simulink model "Bossi_Emanuele_EE460S3D_R99"  (R2025a)
settings: Solver=FixedStepDiscrete  StartTime=0.0  StopTime=120  FixedStep=dt0  RelTol=1e-3  EnableMultiTasking=on
PostLoadFcn:
  | %Set the size for the model
  | set_param(gcs,'Location',[10 10 1270 970])
  | %Set the zoom factor for the model
  | set_param(gcs,'ZoomFactor','100')
InitFcn:
  | tic
  | Bossi_Emanuele_EE460_Final
  | INIT_S3D_01
StartFcn:
  | tend0=toc;
  | tic;
StopFcn:
  | tend=toc;
  | disp(['Simulation time = ' num2str(tout(end)) ' sec'])
  | disp(['Real time = ' num2str(tend) ' sec'])
  | title('DONE')
  | SCORE=round((max(0,120-tout(end)-tend0))*4+10*(40-FuelBurned)+sum(100*double(PDONE)-100*double(PDONE<.5)));
  | PlotS3D(PlotInput);
  | text(15,22,['S: ' num2str(SCORE)]);
  | % Reset color scheme back to normal defaults
  | figure()
  | blkwhitebg('w');
  | close
values from neighbouring files (symbols this model uses):
  A_obs = [ 0  1  0  0  0  0 ... (first row only)    [Bossi_Emanuele_EE460_Final.m]
  B_obs = [ 0     0     0 ... (first row only)    [Bossi_Emanuele_EE460_Final.m]
  C_obs = [ 1 0 0 0 0 0 ... (first row only)    [Bossi_Emanuele_EE460_Final.m]
  d2r = pi/180    (= 0.0174532925199)    [INIT_S3D_01.m]
  D_obs = [ 0     0     0 ... (first row only)    [Bossi_Emanuele_EE460_Final.m]
  dt = 0.01    [INIT_S3D_01.m]
  dt0 = 0.001    [INIT_S3D_01.m]
  fr = 100    [INIT_S3D_01.m]
  G = [1,  1, -1, -1,  0,  0,  0,  0 ... (first row only)    [Bossi_Emanuele_EE460_Final.m]
  G_obs = eye(6)    [Bossi_Emanuele_EE460_Final.m]
  HM_S = 250    [INIT_S3D_01.m]
  HM_U = 500    [INIT_S3D_01.m]
  J = Jbase+JC0+JF+M*(Xcg^2+Ycg^2)    [INIT_S3D_01.m]
  Jbase = JC1+4*Ja+2*Ma*da^2+2*Ma*db^2    [INIT_S3D_01.m]
  JC0 = MC0/2    (= 10.2101761242)    [INIT_S3D_01.m]
  Kdtheta = 2 * zeta_th * wn_th * J_eff    [Bossi_Emanuele_EE460_Final.m]
  Kdtheta_fail = 2 * zeta_th_fail * wn_th_fail * J_eff    [Bossi_Emanuele_EE460_Final.m]
  Kdx = 2 * zeta_xy * wn_xy * M_eff    [Bossi_Emanuele_EE460_Final.m]
  Kdx_fail = 2 * zeta_xy_fail * wn_xy_fail * M_eff    [Bossi_Emanuele_EE460_Final.m]
  Kdy = 2 * zeta_xy * wn_xy * M_eff    [Bossi_Emanuele_EE460_Final.m]
  Kdy_fail = 2 * zeta_xy_fail * wn_xy_fail * M_eff    [Bossi_Emanuele_EE460_Final.m]
  Kptheta = J_eff * wn_th^2    [Bossi_Emanuele_EE460_Final.m]
  Kptheta_fail = J_eff * wn_th_fail^2    [Bossi_Emanuele_EE460_Final.m]
  Kpx = M_eff * wn_xy^2    [Bossi_Emanuele_EE460_Final.m]
  Kpx_fail = M_eff * wn_xy_fail^2    [Bossi_Emanuele_EE460_Final.m]
  Kpy = M_eff * wn_xy^2    [Bossi_Emanuele_EE460_Final.m]
  Kpy_fail = M_eff * wn_xy_fail^2    [Bossi_Emanuele_EE460_Final.m]
  L13 = sqrt(10)    [INIT_S3D_01.m]
  L24 = sqrt(6.25)    [INIT_S3D_01.m]
  LVL = LVL12    [INIT_S3D_01.m]
  M = MC+M1+M2+M3+M4+4*Ma    [INIT_S3D_01.m]
  M1 = LVL.M1    [INIT_S3D_01.m]
  M2 = LVL.M2    [INIT_S3D_01.m]
  M3 = LVL.M3    [INIT_S3D_01.m]
  M4 = LVL.M4    [INIT_S3D_01.m]
  max_qddot = [max_qddot_x; max_qddot_y; max_qddot_theta]    [Bossi_Emanuele_EE460_Final.m]
  mdti = (1/300)    (= 0.00333333333333)    [INIT_S3D_01.m]
  P = [1  1 -1 -1  0  0  0  0 ... (first row only)    [Bossi_Emanuele_EE460_Final.m]
  Pdata = [LVL.P1 LVL.P2 LVL.P3 LVL.P4]    [INIT_S3D_01.m]    (also in PlotS3D.m = R*[xt1;yt1+[0 3*tt*TV(idx-13)*TSIG(idx-13) 0]])
  PTvec = [Pdata(:,1);Pdata(:,2);Pdata(:,3);Pdata(:,4) ... (first row only)    [INIT_S3D_01.m]
  Q_obs = eye(6)    [Bossi_Emanuele_EE460_Final.m]
  r2d = 180/pi    (= 57.2957795131)    [INIT_S3D_01.m]
  r_bang = 0.5    [Bossi_Emanuele_EE460_Final.m]
  Sconfig = 1    [Bossi_Emanuele_EE460_Final.m]
  SLIM = [-100 100 ... (first row only)    [INIT_S3D_01.m]
  SQ = [.005 .01 .004 .005 .01 .004 .02 .01 .4]'    [INIT_S3D_01.m]
  SSF = 1./SQ    [INIT_S3D_01.m]
  tau = 0.5    [Bossi_Emanuele_EE460_Final.m]
  TOLdata = [LVL.P1tol LVL.P2tol LVL.P3tol LVL.P4tol]    [INIT_S3D_01.m]
  ULIM = [[Umin Umax];0 0;0 0]    [INIT_S3D_01.m]
undefined symbols (not defined in the file or in its folder): den_lp, den_lp2, DiscIntNeverNeededParam, dt1_bang_3, dt2_bang_3, dtc_bang_3, num_lp, num_lp2, q0_1
libraries: simulink x87, matrix_library x4, sl3dlib x1, aerolibutil x1, aerolibanimutils x1
(part 7 of 8)

== system Bossi_Emanuele_EE460S3D_R99/S3D_Plant/Sensors/CASE1/THTaccel/CURRENT ==
  In1 : Inport
  Action Port : ActionPort  ActionPortLabel=else
  Out1 : Outport
  wires:
  In1/1 -> Out1/1

== system Bossi_Emanuele_EE460S3D_R99/S3D_Plant/Sensors/CASE1/THTaccel/MAX ==
  Action Port : ActionPort  ActionPortLabel=elseif(u1 > 0.5 & u1 < 1.5)
  Constant : Constant  Value=SLIM(9,2)  SampleTime=dt0
  Out1 : Outport
  wires:
  Constant/1 -> Out1/1

== system Bossi_Emanuele_EE460S3D_R99/S3D_Plant/Sensors/CASE1/THTaccel/MIN ==
  Action Port : ActionPort  ActionPortLabel=if(u1 < -0.5)
  Constant : Constant  Value=SLIM(9,1)  SampleTime=dt0
  Out1 : Outport
  wires:
  Constant/1 -> Out1/1

== system Bossi_Emanuele_EE460S3D_R99/S3D_Plant/Sensors/CASE1/THTpos1/CURRENT ==
  In1 : Inport
  Action Port : ActionPort  ActionPortLabel=else
  Out1 : Outport
  wires:
  In1/1 -> Out1/1

== system Bossi_Emanuele_EE460S3D_R99/S3D_Plant/Sensors/CASE1/THTpos1/MAX ==
  Action Port : ActionPort  ActionPortLabel=elseif(u1 > 0.5 & u1 < 1.5)
  Constant : Constant  Value=SLIM(7,2)  SampleTime=dt0
  Out1 : Outport
  wires:
  Constant/1 -> Out1/1

== system Bossi_Emanuele_EE460S3D_R99/S3D_Plant/Sensors/CASE1/THTpos1/MIN ==
  Action Port : ActionPort  ActionPortLabel=if(u1 < -0.5)
  Constant : Constant  Value=SLIM(7,1)  SampleTime=dt0
  Out1 : Outport
  wires:
  Constant/1 -> Out1/1

== system Bossi_Emanuele_EE460S3D_R99/S3D_Plant/Sensors/CASE1/THTvel/CURRENT ==
  In1 : Inport
  Action Port : ActionPort  ActionPortLabel=else
  Out1 : Outport
  wires:
  In1/1 -> Out1/1

== system Bossi_Emanuele_EE460S3D_R99/S3D_Plant/Sensors/CASE1/THTvel/MAX ==
  Action Port : ActionPort  ActionPortLabel=elseif(u1 > 0.5 & u1 < 1.5)
  Constant : Constant  Value=SLIM(8,2)  SampleTime=dt0
  Out1 : Outport
  wires:
  Constant/1 -> Out1/1

== system Bossi_Emanuele_EE460S3D_R99/S3D_Plant/Sensors/CASE1/THTvel/MIN ==
  Action Port : ActionPort  ActionPortLabel=if(u1 < -0.5)
  Constant : Constant  Value=SLIM(8,1)  SampleTime=dt0
  Out1 : Outport
  wires:
  Constant/1 -> Out1/1

== system Bossi_Emanuele_EE460S3D_R99/S3D_Plant/Sensors/CASE1/Xaccel/CURRENT ==
  In1 : Inport
  Action Port : ActionPort  ActionPortLabel=else
  Out1 : Outport
  wires:
  In1/1 -> Out1/1

== system Bossi_Emanuele_EE460S3D_R99/S3D_Plant/Sensors/CASE1/Xaccel/MAX ==
  Action Port : ActionPort  ActionPortLabel=elseif(u1 > 0.5 & u1 < 1.5)
  Constant : Constant  Value=SLIM(3,2)  SampleTime=dt0
  Out1 : Outport
  wires:
  Constant/1 -> Out1/1

== system Bossi_Emanuele_EE460S3D_R99/S3D_Plant/Sensors/CASE1/Xaccel/MIN ==
  Action Port : ActionPort  ActionPortLabel=if(u1 < -0.5)
  Constant : Constant  Value=SLIM(3,1)  SampleTime=dt0
  Out1 : Outport
  wires:
  Constant/1 -> Out1/1

== system Bossi_Emanuele_EE460S3D_R99/S3D_Plant/Sensors/CASE1/Xpos1/CURRENT ==
  In1 : Inport
  Action Port : ActionPort  ActionPortLabel=else
  Out1 : Outport
  wires:
  In1/1 -> Out1/1

== system Bossi_Emanuele_EE460S3D_R99/S3D_Plant/Sensors/CASE1/Xpos1/MAX ==
  Action Port : ActionPort  ActionPortLabel=elseif(u1 > 0.5 & u1 < 1.5)
  Constant : Constant  Value=SLIM(1,2)  SampleTime=dt0
  Out1 : Outport
  wires:
  Constant/1 -> Out1/1

== system Bossi_Emanuele_EE460S3D_R99/S3D_Plant/Sensors/CASE1/Xpos1/MIN ==
  Action Port : ActionPort  ActionPortLabel=if(u1 < -0.5)
  Constant : Constant  Value=SLIM(1,1)  SampleTime=dt0
  Out1 : Outport
  wires:
  Constant/1 -> Out1/1

== system Bossi_Emanuele_EE460S3D_R99/S3D_Plant/Sensors/CASE1/Xvel/CURRENT ==
  In1 : Inport
  Action Port : ActionPort  ActionPortLabel=else
  Out1 : Outport
  wires:
  In1/1 -> Out1/1

== system Bossi_Emanuele_EE460S3D_R99/S3D_Plant/Sensors/CASE1/Xvel/MAX ==
  Action Port : ActionPort  ActionPortLabel=elseif(u1 > 0.5 & u1 < 1.5)
  Constant : Constant  Value=SLIM(2,2)  SampleTime=dt0
  Out1 : Outport
  wires:
  Constant/1 -> Out1/1

== system Bossi_Emanuele_EE460S3D_R99/S3D_Plant/Sensors/CASE1/Xvel/MIN ==
  Action Port : ActionPort  ActionPortLabel=if(u1 < -0.5)
  Constant : Constant  Value=SLIM(2,1)  SampleTime=dt0
  Out1 : Outport
  wires:
  Constant/1 -> Out1/1

== system Bossi_Emanuele_EE460S3D_R99/S3D_Plant/Sensors/CASE1/Yaccel/CURRENT ==
  In1 : Inport
  Action Port : ActionPort  ActionPortLabel=else
  Out1 : Outport
  wires:
  In1/1 -> Out1/1

== system Bossi_Emanuele_EE460S3D_R99/S3D_Plant/Sensors/CASE1/Yaccel/MAX ==
  Action Port : ActionPort  ActionPortLabel=elseif(u1 > 0.5 & u1 < 1.5)
  Constant : Constant  Value=SLIM(6,2)  SampleTime=dt0
  Out1 : Outport
  wires:
  Constant/1 -> Out1/1

== system Bossi_Emanuele_EE460S3D_R99/S3D_Plant/Sensors/CASE1/Yaccel/MIN ==
  Action Port : ActionPort  ActionPortLabel=if(u1 < -0.5)
  Constant : Constant  Value=SLIM(6,1)  SampleTime=dt0
  Out1 : Outport
  wires:
  Constant/1 -> Out1/1

== system Bossi_Emanuele_EE460S3D_R99/S3D_Plant/Sensors/CASE1/Ypos1/CURRENT ==
  In1 : Inport
  Action Port : ActionPort  ActionPortLabel=else
  Out1 : Outport
  wires:
  In1/1 -> Out1/1

== system Bossi_Emanuele_EE460S3D_R99/S3D_Plant/Sensors/CASE1/Ypos1/MAX ==
  Action Port : ActionPort  ActionPortLabel=elseif(u1 > 0.5 & u1 < 1.5)
  Constant : Constant  Value=SLIM(4,2)  SampleTime=dt0
  Out1 : Outport
  wires:
  Constant/1 -> Out1/1

== system Bossi_Emanuele_EE460S3D_R99/S3D_Plant/Sensors/CASE1/Ypos1/MIN ==
  Action Port : ActionPort  ActionPortLabel=if(u1 < -0.5)
  Constant : Constant  Value=SLIM(4,1)  SampleTime=dt0
  Out1 : Outport
  wires:
  Constant/1 -> Out1/1

== system Bossi_Emanuele_EE460S3D_R99/S3D_Plant/Sensors/CASE1/Yvel/CURRENT ==
  In1 : Inport
  Action Port : ActionPort  ActionPortLabel=else
  Out1 : Outport
  wires:
  In1/1 -> Out1/1

== system Bossi_Emanuele_EE460S3D_R99/S3D_Plant/Sensors/CASE1/Yvel/MAX ==
  Action Port : ActionPort  ActionPortLabel=elseif(u1 > 0.5 & u1 < 1.5)
  Constant : Constant  Value=SLIM(5,2)  SampleTime=dt0
  Out1 : Outport
  wires:
  Constant/1 -> Out1/1

== system Bossi_Emanuele_EE460S3D_R99/S3D_Plant/Sensors/CASE1/Yvel/MIN ==
  Action Port : ActionPort  ActionPortLabel=if(u1 < -0.5)
  Constant : Constant  Value=SLIM(5,1)  SampleTime=dt0
  Out1 : Outport
  wires:
  Constant/1 -> Out1/1

== system Bossi_Emanuele_EE460S3D_R99/S3D_Plant/Sensors/CASE2/THTpos1/CURRENT ==
  In1 : Inport
  Action Port : ActionPort  ActionPortLabel=else
  Out1 : Outport
  wires:
  In1/1 -> Out1/1

== system Bossi_Emanuele_EE460S3D_R99/S3D_Plant/Sensors/CASE2/THTpos1/MAX ==
  Action Port : ActionPort  ActionPortLabel=elseif(u1 > 0.5 & u1 < 1.5)
  Constant : Constant  Value=SLIM(7,2)  SampleTime=dt0
  Out1 : Outport
  wires:
  Constant/1 -> Out1/1

== system Bossi_Emanuele_EE460S3D_R99/S3D_Plant/Sensors/CASE2/THTpos1/MIN ==
  Action Port : ActionPort  ActionPortLabel=if(u1 < -0.5)
  Constant : Constant  Value=SLIM(7,1)  SampleTime=dt0
  Out1 : Outport
  wires:
  Constant/1 -> Out1/1

== system Bossi_Emanuele_EE460S3D_R99/S3D_Plant/Sensors/CASE2/THTpos2/CURRENT ==
  In1 : Inport
  Action Port : ActionPort  ActionPortLabel=else
  Out1 : Outport
  wires:
  In1/1 -> Out1/1

== system Bossi_Emanuele_EE460S3D_R99/S3D_Plant/Sensors/CASE2/THTpos2/MAX ==
  Action Port : ActionPort  ActionPortLabel=elseif(u1 > 0.5 & u1 < 1.5)
  Constant : Constant  Value=SLIM(7,2)  SampleTime=dt0
  Out1 : Outport
  wires:
  Constant/1 -> Out1/1

== system Bossi_Emanuele_EE460S3D_R99/S3D_Plant/Sensors/CASE2/THTpos2/MIN ==
  Action Port : ActionPort  ActionPortLabel=if(u1 < -0.5)
  Constant : Constant  Value=SLIM(7,1)  SampleTime=dt0
  Out1 : Outport
  wires:
  Constant/1 -> Out1/1

== system Bossi_Emanuele_EE460S3D_R99/S3D_Plant/Sensors/CASE2/THTvel/CURRENT ==
  In1 : Inport
  Action Port : ActionPort  ActionPortLabel=else
  Out1 : Outport
  wires:
  In1/1 -> Out1/1

== system Bossi_Emanuele_EE460S3D_R99/S3D_Plant/Sensors/CASE2/THTvel/MAX ==
  Action Port : ActionPort  ActionPortLabel=elseif(u1 > 0.5 & u1 < 1.5)
  Constant : Constant  Value=SLIM(8,2)  SampleTime=dt0
  Out1 : Outport
  wires:
  Constant/1 -> Out1/1

== system Bossi_Emanuele_EE460S3D_R99/S3D_Plant/Sensors/CASE2/THTvel/MIN ==
  Action Port : ActionPort  ActionPortLabel=if(u1 < -0.5)
  Constant : Constant  Value=SLIM(8,1)  SampleTime=dt0
  Out1 : Outport
  wires:
  Constant/1 -> Out1/1

== system Bossi_Emanuele_EE460S3D_R99/S3D_Plant/Sensors/CASE2/Xpos1/CURRENT ==
  In1 : Inport
  Action Port : ActionPort  ActionPortLabel=else
  Out1 : Outport
  wires:
  In1/1 -> Out1/1

== system Bossi_Emanuele_EE460S3D_R99/S3D_Plant/Sensors/CASE2/Xpos1/MAX ==
  Action Port : ActionPort  ActionPortLabel=elseif(u1 > 0.5 & u1 < 1.5)
  Constant : Constant  Value=SLIM(1,2)  SampleTime=dt0
  Out1 : Outport
  wires:
  Constant/1 -> Out1/1

== system Bossi_Emanuele_EE460S3D_R99/S3D_Plant/Sensors/CASE2/Xpos1/MIN ==
  Action Port : ActionPort  ActionPortLabel=if(u1 < -0.5)
  Constant : Constant  Value=SLIM(1,1)  SampleTime=dt0
  Out1 : Outport
  wires:
  Constant/1 -> Out1/1

== system Bossi_Emanuele_EE460S3D_R99/S3D_Plant/Sensors/CASE2/Xpos2/CURRENT ==
  In1 : Inport
  Action Port : ActionPort  ActionPortLabel=else
  Out1 : Outport
  wires:
  In1/1 -> Out1/1

== system Bossi_Emanuele_EE460S3D_R99/S3D_Plant/Sensors/CASE2/Xpos2/MAX ==
  Action Port : ActionPort  ActionPortLabel=elseif(u1 > 0.5 & u1 < 1.5)
  Constant : Constant  Value=SLIM(1,2)  SampleTime=dt0
  Out1 : Outport
  wires:
  Constant/1 -> Out1/1

== system Bossi_Emanuele_EE460S3D_R99/S3D_Plant/Sensors/CASE2/Xpos2/MIN ==
  Action Port : ActionPort  ActionPortLabel=if(u1 < -0.5)
  Constant : Constant  Value=SLIM(1,1)  SampleTime=dt0
  Out1 : Outport
  wires:
  Constant/1 -> Out1/1

== system Bossi_Emanuele_EE460S3D_R99/S3D_Plant/Sensors/CASE2/Xvel/CURRENT ==
  In1 : Inport
  Action Port : ActionPort  ActionPortLabel=else
  Out1 : Outport
  wires:
  In1/1 -> Out1/1

== system Bossi_Emanuele_EE460S3D_R99/S3D_Plant/Sensors/CASE2/Xvel/MAX ==
  Action Port : ActionPort  ActionPortLabel=elseif(u1 > 0.5 & u1 < 1.5)
  Constant : Constant  Value=SLIM(2,2)  SampleTime=dt0
  Out1 : Outport
  wires:
  Constant/1 -> Out1/1

== system Bossi_Emanuele_EE460S3D_R99/S3D_Plant/Sensors/CASE2/Xvel/MIN ==
  Action Port : ActionPort  ActionPortLabel=if(u1 < -0.5)
  Constant : Constant  Value=SLIM(2,1)  SampleTime=dt0
  Out1 : Outport
  wires:
  Constant/1 -> Out1/1

== system Bossi_Emanuele_EE460S3D_R99/S3D_Plant/Sensors/CASE2/Ypos1/CURRENT ==
  In1 : Inport
  Action Port : ActionPort  ActionPortLabel=else
  Out1 : Outport
  wires:
  In1/1 -> Out1/1

== system Bossi_Emanuele_EE460S3D_R99/S3D_Plant/Sensors/CASE2/Ypos1/MAX ==
  Action Port : ActionPort  ActionPortLabel=elseif(u1 > 0.5 & u1 < 1.5)
  Constant : Constant  Value=SLIM(4,2)  SampleTime=dt0
  Out1 : Outport
  wires:
  Constant/1 -> Out1/1

== system Bossi_Emanuele_EE460S3D_R99/S3D_Plant/Sensors/CASE2/Ypos1/MIN ==
  Action Port : ActionPort  ActionPortLabel=if(u1 < -0.5)
  Constant : Constant  Value=SLIM(4,1)  SampleTime=dt0
  Out1 : Outport
  wires:
  Constant/1 -> Out1/1

== system Bossi_Emanuele_EE460S3D_R99/S3D_Plant/Sensors/CASE2/Ypos2/CURRENT ==
  In1 : Inport
  Action Port : ActionPort  ActionPortLabel=else
  Out1 : Outport
  wires:
  In1/1 -> Out1/1

== system Bossi_Emanuele_EE460S3D_R99/S3D_Plant/Sensors/CASE2/Ypos2/MAX ==
  Action Port : ActionPort  ActionPortLabel=elseif(u1 > 0.5 & u1 < 1.5)
  Constant : Constant  Value=SLIM(4,2)  SampleTime=dt0
  Out1 : Outport
  wires:
  Constant/1 -> Out1/1

== system Bossi_Emanuele_EE460S3D_R99/S3D_Plant/Sensors/CASE2/Ypos2/MIN ==
  Action Port : ActionPort  ActionPortLabel=if(u1 < -0.5)
  Constant : Constant  Value=SLIM(4,1)  SampleTime=dt0
  Out1 : Outport
  wires:
  Constant/1 -> Out1/1

== system Bossi_Emanuele_EE460S3D_R99/S3D_Plant/Sensors/CASE2/Yvel/CURRENT ==
  In1 : Inport
  Action Port : ActionPort  ActionPortLabel=else
  Out1 : Outport
  wires:
  In1/1 -> Out1/1

== system Bossi_Emanuele_EE460S3D_R99/S3D_Plant/Sensors/CASE2/Yvel/MAX ==
  Action Port : ActionPort  ActionPortLabel=elseif(u1 > 0.5 & u1 < 1.5)
  Constant : Constant  Value=SLIM(5,2)  SampleTime=dt0
  Out1 : Outport
  wires:
  Constant/1 -> Out1/1

== system Bossi_Emanuele_EE460S3D_R99/S3D_Plant/Sensors/CASE2/Yvel/MIN ==
  Action Port : ActionPort  ActionPortLabel=if(u1 < -0.5)
  Constant : Constant  Value=SLIM(5,1)  SampleTime=dt0
  Out1 : Outport
  wires:
  Constant/1 -> Out1/1

== system Bossi_Emanuele_EE460S3D_R99/S3D_Plant/Sensors/CASE3/THTpos1/CURRENT ==
  In1 : Inport
  Action Port : ActionPort  ActionPortLabel=else
  Out1 : Outport
  wires:
  In1/1 -> Out1/1

== system Bossi_Emanuele_EE460S3D_R99/S3D_Plant/Sensors/CASE3/THTpos1/MAX ==
  Action Port : ActionPort  ActionPortLabel=elseif(u1 > 0.5 & u1 < 1.5)
  Constant : Constant  Value=SLIM(7,2)  SampleTime=dt0
  Out1 : Outport
  wires:
  Constant/1 -> Out1/1

== system Bossi_Emanuele_EE460S3D_R99/S3D_Plant/Sensors/CASE3/THTpos1/MIN ==
  Action Port : ActionPort  ActionPortLabel=if(u1 < -0.5)
  Constant : Constant  Value=SLIM(7,1)  SampleTime=dt0
  Out1 : Outport
  wires:
  Constant/1 -> Out1/1

== system Bossi_Emanuele_EE460S3D_R99/S3D_Plant/Sensors/CASE3/THTpos2/CURRENT ==
  In1 : Inport
  Action Port : ActionPort  ActionPortLabel=else
  Out1 : Outport
  wires:
  In1/1 -> Out1/1

== system Bossi_Emanuele_EE460S3D_R99/S3D_Plant/Sensors/CASE3/THTpos2/MAX ==
  Action Port : ActionPort  ActionPortLabel=elseif(u1 > 0.5 & u1 < 1.5)
  Constant : Constant  Value=SLIM(7,2)  SampleTime=dt0
  Out1 : Outport
  wires:
  Constant/1 -> Out1/1

== system Bossi_Emanuele_EE460S3D_R99/S3D_Plant/Sensors/CASE3/THTpos2/MIN ==
  Action Port : ActionPort  ActionPortLabel=if(u1 < -0.5)
  Constant : Constant  Value=SLIM(7,1)  SampleTime=dt0
  Out1 : Outport
  wires:
  Constant/1 -> Out1/1

== system Bossi_Emanuele_EE460S3D_R99/S3D_Plant/Sensors/CASE3/THTpos3/CURRENT ==
  In1 : Inport
  Action Port : ActionPort  ActionPortLabel=else
  Out1 : Outport
  wires:
  In1/1 -> Out1/1

== system Bossi_Emanuele_EE460S3D_R99/S3D_Plant/Sensors/CASE3/THTpos3/MAX ==
  Action Port : ActionPort  ActionPortLabel=elseif(u1 > 0.5 & u1 < 1.5)
  Constant : Constant  Value=SLIM(7,2)  SampleTime=dt0
  Out1 : Outport
  wires:
  Constant/1 -> Out1/1

== system Bossi_Emanuele_EE460S3D_R99/S3D_Plant/Sensors/CASE3/THTpos3/MIN ==
  Action Port : ActionPort  ActionPortLabel=if(u1 < -0.5)
  Constant : Constant  Value=SLIM(7,1)  SampleTime=dt0
  Out1 : Outport
  wires:
  Constant/1 -> Out1/1

== system Bossi_Emanuele_EE460S3D_R99/S3D_Plant/Sensors/CASE3/Xpos1/CURRENT ==
  In1 : Inport
  Action Port : ActionPort  ActionPortLabel=else
  Out1 : Outport
  wires:
  In1/1 -> Out1/1

== system Bossi_Emanuele_EE460S3D_R99/S3D_Plant/Sensors/CASE3/Xpos1/MAX ==
  Action Port : ActionPort  ActionPortLabel=elseif(u1 > 0.5 & u1 < 1.5)
  Constant : Constant  Value=SLIM(1,2)  SampleTime=dt0
  Out1 : Outport
  wires:
  Constant/1 -> Out1/1

== system Bossi_Emanuele_EE460S3D_R99/S3D_Plant/Sensors/CASE3/Xpos1/MIN ==
  Action Port : ActionPort  ActionPortLabel=if(u1 < -0.5)
  Constant : Constant  Value=SLIM(1,1)  SampleTime=dt0
  Out1 : Outport
  wires:
  Constant/1 -> Out1/1

== system Bossi_Emanuele_EE460S3D_R99/S3D_Plant/Sensors/CASE3/Xpos2/CURRENT ==
  In1 : Inport
  Action Port : ActionPort  ActionPortLabel=else
  Out1 : Outport
  wires:
  In1/1 -> Out1/1

== system Bossi_Emanuele_EE460S3D_R99/S3D_Plant/Sensors/CASE3/Xpos2/MAX ==
  Action Port : ActionPort  ActionPortLabel=elseif(u1 > 0.5 & u1 < 1.5)
  Constant : Constant  Value=SLIM(1,2)  SampleTime=dt0
  Out1 : Outport
  wires:
  Constant/1 -> Out1/1

== system Bossi_Emanuele_EE460S3D_R99/S3D_Plant/Sensors/CASE3/Xpos2/MIN ==
  Action Port : ActionPort  ActionPortLabel=if(u1 < -0.5)
  Constant : Constant  Value=SLIM(1,1)  SampleTime=dt0
  Out1 : Outport
  wires:
  Constant/1 -> Out1/1

== system Bossi_Emanuele_EE460S3D_R99/S3D_Plant/Sensors/CASE3/Xpos3/CURRENT ==
  In1 : Inport
  Action Port : ActionPort  ActionPortLabel=else
  Out1 : Outport
  wires:
  In1/1 -> Out1/1

== system Bossi_Emanuele_EE460S3D_R99/S3D_Plant/Sensors/CASE3/Xpos3/MAX ==
  Action Port : ActionPort  ActionPortLabel=elseif(u1 > 0.5 & u1 < 1.5)
  Constant : Constant  Value=SLIM(1,2)  SampleTime=dt0
  Out1 : Outport
  wires:
  Constant/1 -> Out1/1

== system Bossi_Emanuele_EE460S3D_R99/S3D_Plant/Sensors/CASE3/Xpos3/MIN ==
  Action Port : ActionPort  ActionPortLabel=if(u1 < -0.5)
  Constant : Constant  Value=SLIM(1,1)  SampleTime=dt0
  Out1 : Outport
  wires:
  Constant/1 -> Out1/1

== system Bossi_Emanuele_EE460S3D_R99/S3D_Plant/Sensors/CASE3/Ypos1/CURRENT ==
  In1 : Inport
  Action Port : ActionPort  ActionPortLabel=else
  Out1 : Outport
  wires:
  In1/1 -> Out1/1

== system Bossi_Emanuele_EE460S3D_R99/S3D_Plant/Sensors/CASE3/Ypos1/MAX ==
  Action Port : ActionPort  ActionPortLabel=elseif(u1 > 0.5 & u1 < 1.5)
  Constant : Constant  Value=SLIM(4,2)  SampleTime=dt0
  Out1 : Outport
  wires:
  Constant/1 -> Out1/1

== system Bossi_Emanuele_EE460S3D_R99/S3D_Plant/Sensors/CASE3/Ypos1/MIN ==
  Action Port : ActionPort  ActionPortLabel=if(u1 < -0.5)
  Constant : Constant  Value=SLIM(4,1)  SampleTime=dt0
  Out1 : Outport
  wires:
  Constant/1 -> Out1/1

== system Bossi_Emanuele_EE460S3D_R99/S3D_Plant/Sensors/CASE3/Ypos2/CURRENT ==
  In1 : Inport
  Action Port : ActionPort  ActionPortLabel=else
  Out1 : Outport
  wires:
  In1/1 -> Out1/1

== system Bossi_Emanuele_EE460S3D_R99/S3D_Plant/Sensors/CASE3/Ypos2/MAX ==
  Action Port : ActionPort  ActionPortLabel=elseif(u1 > 0.5 & u1 < 1.5)
  Constant : Constant  Value=SLIM(4,2)  SampleTime=dt0
  Out1 : Outport
  wires:
  Constant/1 -> Out1/1

== system Bossi_Emanuele_EE460S3D_R99/S3D_Plant/Sensors/CASE3/Ypos2/MIN ==
  Action Port : ActionPort  ActionPortLabel=if(u1 < -0.5)
  Constant : Constant  Value=SLIM(4,1)  SampleTime=dt0
  Out1 : Outport
  wires:
  Constant/1 -> Out1/1

== system Bossi_Emanuele_EE460S3D_R99/S3D_Plant/Sensors/CASE3/Ypos3/CURRENT ==
  In1 : Inport
  Action Port : ActionPort  ActionPortLabel=else
  Out1 : Outport
  wires:
  In1/1 -> Out1/1

== system Bossi_Emanuele_EE460S3D_R99/S3D_Plant/Sensors/CASE3/Ypos3/MAX ==
  Action Port : ActionPort  ActionPortLabel=elseif(u1 > 0.5 & u1 < 1.5)
  Constant : Constant  Value=SLIM(4,2)  SampleTime=dt0
  Out1 : Outport
  wires:
  Constant/1 -> Out1/1

== system Bossi_Emanuele_EE460S3D_R99/S3D_Plant/Sensors/CASE3/Ypos3/MIN ==
  Action Port : ActionPort  ActionPortLabel=if(u1 < -0.5)
  Constant : Constant  Value=SLIM(4,1)  SampleTime=dt0
  Out1 : Outport
  wires:
  Constant/1 -> Out1/1

== system Bossi_Emanuele_EE460S3D_R99/S3D_Plant/ThrusterValues/FailModes/Ufail1/CURRENT ==
  In1 : Inport
  Action Port : ActionPort  ActionPortLabel=else
  Out1 : Outport
  wires:
  In1/1 -> Out1/1

== system Bossi_Emanuele_EE460S3D_R99/S3D_Plant/ThrusterValues/FailModes/Ufail1/FailLogic ==
  BeforeFail : Inport
  FuelRemaining : Inport  Port=2
  FailMode : Inport  Port=3
  Abs : Abs  SaturateOnIntegerOverflow=off
  Compare To Constant : simulink/Logic and Bit Operations/Compare To Constant  relop=<=  const=0.5  OutDataTypeStr=boolean
  Logical Operator : Logic  Operator=OR  AllPortsSameDT=off  OutDataTypeStr=boolean
  Logical Operator1 : Logic  AllPortsSameDT=off  OutDataTypeStr=boolean
  NoFail : Outport
  wires:
  FailMode/1 -> Abs/1
  Logical Operator1/1 -> NoFail/1
  Compare To Constant/1 -> Logical Operator/2
  BeforeFail/1 -> Logical Operator/1
  Abs/1 -> Compare To Constant/1
  Logical Operator/1 -> Logical Operator1/1
  FuelRemaining/1 -> Logical Operator1/2

== system Bossi_Emanuele_EE460S3D_R99/S3D_Plant/ThrusterValues/FailModes/Ufail1/MAX ==
  Action Port : ActionPort  ActionPortLabel=elseif(u1 > 0.5 & u1 < 1.5)
  Constant : Constant  Value=ULIM(Udx,2)  SampleTime=dt0
  Out1 : Outport
  wires:
  Constant/1 -> Out1/1

== system Bossi_Emanuele_EE460S3D_R99/S3D_Plant/ThrusterValues/FailModes/Ufail1/MIN ==
  Action Port : ActionPort  ActionPortLabel=if(u1 < -0.5)
  Constant : Constant  Value=ULIM(Udx,1)  SampleTime=dt0
  Out1 : Outport
  wires:
  Constant/1 -> Out1/1

== system Bossi_Emanuele_EE460S3D_R99/S3D_Plant/ThrusterValues/FailModes/Ufail10/CURRENT ==
  In1 : Inport
  Action Port : ActionPort  ActionPortLabel=else
  Out1 : Outport
  wires:
  In1/1 -> Out1/1

== system Bossi_Emanuele_EE460S3D_R99/S3D_Plant/ThrusterValues/FailModes/Ufail10/FailLogic ==
  BeforeFail : Inport
  FuelRemaining : Inport  Port=2
  FailMode : Inport  Port=3
  Abs : Abs  SaturateOnIntegerOverflow=off
  Compare To Constant : simulink/Logic and Bit Operations/Compare To Constant  relop=<=  const=0.5  OutDataTypeStr=boolean
  Logical Operator : Logic  Operator=OR  AllPortsSameDT=off  OutDataTypeStr=boolean
  Logical Operator1 : Logic  AllPortsSameDT=off  OutDataTypeStr=boolean
  NoFail : Outport
  wires:
  FailMode/1 -> Abs/1
  Logical Operator1/1 -> NoFail/1
  Compare To Constant/1 -> Logical Operator/2
  BeforeFail/1 -> Logical Operator/1
  Abs/1 -> Compare To Constant/1
  Logical Operator/1 -> Logical Operator1/1
  FuelRemaining/1 -> Logical Operator1/2

== system Bossi_Emanuele_EE460S3D_R99/S3D_Plant/ThrusterValues/FailModes/Ufail10/MAX ==
  Action Port : ActionPort  ActionPortLabel=elseif(u1 > 0.5 & u1 < 1.5)
  Constant : Constant  Value=ULIM(Udx,2)  SampleTime=dt0
  Out1 : Outport
  wires:
  Constant/1 -> Out1/1

== system Bossi_Emanuele_EE460S3D_R99/S3D_Plant/ThrusterValues/FailModes/Ufail10/MIN ==
  Action Port : ActionPort  ActionPortLabel=if(u1 < -0.5)
  Constant : Constant  Value=ULIM(Udx,1)  SampleTime=dt0
  Out1 : Outport
  wires:
  Constant/1 -> Out1/1

== system Bossi_Emanuele_EE460S3D_R99/S3D_Plant/ThrusterValues/FailModes/Ufail2/CURRENT ==
  In1 : Inport
  Action Port : ActionPort  ActionPortLabel=else
  Out1 : Outport
  wires:
  In1/1 -> Out1/1

== system Bossi_Emanuele_EE460S3D_R99/S3D_Plant/ThrusterValues/FailModes/Ufail2/FailLogic ==
  BeforeFail : Inport
  FuelRemaining : Inport  Port=2
  FailMode : Inport  Port=3
  Abs : Abs  SaturateOnIntegerOverflow=off
  Compare To Constant : simulink/Logic and Bit Operations/Compare To Constant  relop=<=  const=0.5  OutDataTypeStr=boolean
  Logical Operator : Logic  Operator=OR  AllPortsSameDT=off  OutDataTypeStr=boolean
  Logical Operator1 : Logic  AllPortsSameDT=off  OutDataTypeStr=boolean
  NoFail : Outport
  wires:
  FailMode/1 -> Abs/1
  Logical Operator1/1 -> NoFail/1
  Compare To Constant/1 -> Logical Operator/2
  BeforeFail/1 -> Logical Operator/1
  Abs/1 -> Compare To Constant/1
  Logical Operator/1 -> Logical Operator1/1
  FuelRemaining/1 -> Logical Operator1/2

== system Bossi_Emanuele_EE460S3D_R99/S3D_Plant/ThrusterValues/FailModes/Ufail2/MAX ==
  Action Port : ActionPort  ActionPortLabel=elseif(u1 > 0.5 & u1 < 1.5)
  Constant : Constant  Value=ULIM(Udx,2)  SampleTime=dt0
  Out1 : Outport
  wires:
  Constant/1 -> Out1/1

== system Bossi_Emanuele_EE460S3D_R99/S3D_Plant/ThrusterValues/FailModes/Ufail2/MIN ==
  Action Port : ActionPort  ActionPortLabel=if(u1 < -0.5)
  Constant : Constant  Value=ULIM(Udx,1)  SampleTime=dt0
  Out1 : Outport
  wires:
  Constant/1 -> Out1/1

== system Bossi_Emanuele_EE460S3D_R99/S3D_Plant/ThrusterValues/FailModes/Ufail3/CURRENT ==
  In1 : Inport
  Action Port : ActionPort  ActionPortLabel=else
  Out1 : Outport
  wires:
  In1/1 -> Out1/1

== system Bossi_Emanuele_EE460S3D_R99/S3D_Plant/ThrusterValues/FailModes/Ufail3/FailLogic ==
  BeforeFail : Inport
  FuelRemaining : Inport  Port=2
  FailMode : Inport  Port=3
  Abs : Abs  SaturateOnIntegerOverflow=off
  Compare To Constant : simulink/Logic and Bit Operations/Compare To Constant  relop=<=  const=0.5  OutDataTypeStr=boolean
  Logical Operator : Logic  Operator=OR  AllPortsSameDT=off  OutDataTypeStr=boolean
  Logical Operator1 : Logic  AllPortsSameDT=off  OutDataTypeStr=boolean
  NoFail : Outport
  wires:
  FailMode/1 -> Abs/1
  Logical Operator1/1 -> NoFail/1
  Compare To Constant/1 -> Logical Operator/2
  BeforeFail/1 -> Logical Operator/1
  Abs/1 -> Compare To Constant/1
  Logical Operator/1 -> Logical Operator1/1
  FuelRemaining/1 -> Logical Operator1/2

== system Bossi_Emanuele_EE460S3D_R99/S3D_Plant/ThrusterValues/FailModes/Ufail3/MAX ==
  Action Port : ActionPort  ActionPortLabel=elseif(u1 > 0.5 & u1 < 1.5)
  Constant : Constant  Value=ULIM(Udx,2)  SampleTime=dt0
  Out1 : Outport
  wires:
  Constant/1 -> Out1/1

== system Bossi_Emanuele_EE460S3D_R99/S3D_Plant/ThrusterValues/FailModes/Ufail3/MIN ==
  Action Port : ActionPort  ActionPortLabel=if(u1 < -0.5)
  Constant : Constant  Value=ULIM(Udx,1)  SampleTime=dt0
  Out1 : Outport
  wires:
  Constant/1 -> Out1/1

== system Bossi_Emanuele_EE460S3D_R99/S3D_Plant/ThrusterValues/FailModes/Ufail4/CURRENT ==
  In1 : Inport
  Action Port : ActionPort  ActionPortLabel=else
  Out1 : Outport
  wires:
  In1/1 -> Out1/1

== system Bossi_Emanuele_EE460S3D_R99/S3D_Plant/ThrusterValues/FailModes/Ufail4/FailLogic ==
  BeforeFail : Inport
  FuelRemaining : Inport  Port=2
  FailMode : Inport  Port=3
  Abs : Abs  SaturateOnIntegerOverflow=off
  Compare To Constant : simulink/Logic and Bit Operations/Compare To Constant  relop=<=  const=0.5  OutDataTypeStr=boolean
  Logical Operator : Logic  Operator=OR  AllPortsSameDT=off  OutDataTypeStr=boolean
  Logical Operator1 : Logic  AllPortsSameDT=off  OutDataTypeStr=boolean
  NoFail : Outport
  wires:
  FailMode/1 -> Abs/1
  Logical Operator1/1 -> NoFail/1
  Compare To Constant/1 -> Logical Operator/2
  BeforeFail/1 -> Logical Operator/1
  Abs/1 -> Compare To Constant/1
  Logical Operator/1 -> Logical Operator1/1
  FuelRemaining/1 -> Logical Operator1/2

== system Bossi_Emanuele_EE460S3D_R99/S3D_Plant/ThrusterValues/FailModes/Ufail4/MAX ==
  Action Port : ActionPort  ActionPortLabel=elseif(u1 > 0.5 & u1 < 1.5)
  Constant : Constant  Value=ULIM(Udx,2)  SampleTime=dt0
  Out1 : Outport
  wires:
  Constant/1 -> Out1/1

== system Bossi_Emanuele_EE460S3D_R99/S3D_Plant/ThrusterValues/FailModes/Ufail4/MIN ==
  Action Port : ActionPort  ActionPortLabel=if(u1 < -0.5)
  Constant : Constant  Value=ULIM(Udx,1)  SampleTime=dt0
  Out1 : Outport
  wires:
  Constant/1 -> Out1/1

== system Bossi_Emanuele_EE460S3D_R99/S3D_Plant/ThrusterValues/FailModes/Ufail5/CURRENT ==
  In1 : Inport
  Action Port : ActionPort  ActionPortLabel=else
  Out1 : Outport
  wires:
  In1/1 -> Out1/1

== system Bossi_Emanuele_EE460S3D_R99/S3D_Plant/ThrusterValues/FailModes/Ufail5/FailLogic ==
  BeforeFail : Inport
  FuelRemaining : Inport  Port=2
  FailMode : Inport  Port=3
  Abs : Abs  SaturateOnIntegerOverflow=off
  Compare To Constant : simulink/Logic and Bit Operations/Compare To Constant  relop=<=  const=0.5  OutDataTypeStr=boolean
  Logical Operator : Logic  Operator=OR  AllPortsSameDT=off  OutDataTypeStr=boolean
  Logical Operator1 : Logic  AllPortsSameDT=off  OutDataTypeStr=boolean
  NoFail : Outport
  wires:
  FailMode/1 -> Abs/1
  Logical Operator1/1 -> NoFail/1
  Compare To Constant/1 -> Logical Operator/2
  BeforeFail/1 -> Logical Operator/1
  Abs/1 -> Compare To Constant/1
  Logical Operator/1 -> Logical Operator1/1
  FuelRemaining/1 -> Logical Operator1/2

== system Bossi_Emanuele_EE460S3D_R99/S3D_Plant/ThrusterValues/FailModes/Ufail5/MAX ==
  Action Port : ActionPort  ActionPortLabel=elseif(u1 > 0.5 & u1 < 1.5)
  Constant : Constant  Value=ULIM(Udx,2)  SampleTime=dt0
  Out1 : Outport
  wires:
  Constant/1 -> Out1/1

== system Bossi_Emanuele_EE460S3D_R99/S3D_Plant/ThrusterValues/FailModes/Ufail5/MIN ==
  Action Port : ActionPort  ActionPortLabel=if(u1 < -0.5)
  Constant : Constant  Value=ULIM(Udx,1)  SampleTime=dt0
  Out1 : Outport
  wires:
  Constant/1 -> Out1/1

== system Bossi_Emanuele_EE460S3D_R99/S3D_Plant/ThrusterValues/FailModes/Ufail6/CURRENT ==
  In1 : Inport
  Action Port : ActionPort  ActionPortLabel=else
  Out1 : Outport
  wires:
  In1/1 -> Out1/1

== system Bossi_Emanuele_EE460S3D_R99/S3D_Plant/ThrusterValues/FailModes/Ufail6/FailLogic ==
  BeforeFail : Inport
  FuelRemaining : Inport  Port=2
  FailMode : Inport  Port=3
  Abs : Abs  SaturateOnIntegerOverflow=off
  Compare To Constant : simulink/Logic and Bit Operations/Compare To Constant  relop=<=  const=0.5  OutDataTypeStr=boolean
  Logical Operator : Logic  Operator=OR  AllPortsSameDT=off  OutDataTypeStr=boolean
  Logical Operator1 : Logic  AllPortsSameDT=off  OutDataTypeStr=boolean
  NoFail : Outport
  wires:
  FailMode/1 -> Abs/1
  Logical Operator1/1 -> NoFail/1
  Compare To Constant/1 -> Logical Operator/2
  BeforeFail/1 -> Logical Operator/1
  Abs/1 -> Compare To Constant/1
  Logical Operator/1 -> Logical Operator1/1
  FuelRemaining/1 -> Logical Operator1/2

== system Bossi_Emanuele_EE460S3D_R99/S3D_Plant/ThrusterValues/FailModes/Ufail6/MAX ==
  Action Port : ActionPort  ActionPortLabel=elseif(u1 > 0.5 & u1 < 1.5)
  Constant : Constant  Value=ULIM(Udx,2)  SampleTime=dt0
  Out1 : Outport
  wires:
  Constant/1 -> Out1/1

== system Bossi_Emanuele_EE460S3D_R99/S3D_Plant/ThrusterValues/FailModes/Ufail6/MIN ==
  Action Port : ActionPort  ActionPortLabel=if(u1 < -0.5)
  Constant : Constant  Value=ULIM(Udx,1)  SampleTime=dt0
  Out1 : Outport
  wires:
  Constant/1 -> Out1/1

== system Bossi_Emanuele_EE460S3D_R99/S3D_Plant/ThrusterValues/FailModes/Ufail7/CURRENT ==
  In1 : Inport
  Action Port : ActionPort  ActionPortLabel=else
  Out1 : Outport
  wires:
  In1/1 -> Out1/1

== system Bossi_Emanuele_EE460S3D_R99/S3D_Plant/ThrusterValues/FailModes/Ufail7/FailLogic ==
  BeforeFail : Inport
  FuelRemaining : Inport  Port=2
  FailMode : Inport  Port=3
  Abs : Abs  SaturateOnIntegerOverflow=off
  Compare To Constant : simulink/Logic and Bit Operations/Compare To Constant  relop=<=  const=0.5  OutDataTypeStr=boolean
  Logical Operator : Logic  Operator=OR  AllPortsSameDT=off  OutDataTypeStr=boolean
  Logical Operator1 : Logic  AllPortsSameDT=off  OutDataTypeStr=boolean
  NoFail : Outport
  wires:
  FailMode/1 -> Abs/1
  Logical Operator1/1 -> NoFail/1
  Compare To Constant/1 -> Logical Operator/2
  BeforeFail/1 -> Logical Operator/1
  Abs/1 -> Compare To Constant/1
  Logical Operator/1 -> Logical Operator1/1
  FuelRemaining/1 -> Logical Operator1/2

== system Bossi_Emanuele_EE460S3D_R99/S3D_Plant/ThrusterValues/FailModes/Ufail7/MAX ==
  Action Port : ActionPort  ActionPortLabel=elseif(u1 > 0.5 & u1 < 1.5)
  Constant : Constant  Value=ULIM(Udx,2)  SampleTime=dt0
  Out1 : Outport
  wires:
  Constant/1 -> Out1/1

== system Bossi_Emanuele_EE460S3D_R99/S3D_Plant/ThrusterValues/FailModes/Ufail7/MIN ==
  Action Port : ActionPort  ActionPortLabel=if(u1 < -0.5)
  Constant : Constant  Value=ULIM(Udx,1)  SampleTime=dt0
  Out1 : Outport
  wires:
  Constant/1 -> Out1/1

== system Bossi_Emanuele_EE460S3D_R99/S3D_Plant/ThrusterValues/FailModes/Ufail8/CURRENT ==
  In1 : Inport
  Action Port : ActionPort  ActionPortLabel=else
  Out1 : Outport
  wires:
  In1/1 -> Out1/1

== system Bossi_Emanuele_EE460S3D_R99/S3D_Plant/ThrusterValues/FailModes/Ufail8/FailLogic ==
  BeforeFail : Inport
  FuelRemaining : Inport  Port=2
  FailMode : Inport  Port=3
  Abs : Abs  SaturateOnIntegerOverflow=off
  Compare To Constant : simulink/Logic and Bit Operations/Compare To Constant  relop=<=  const=0.5  OutDataTypeStr=boolean
  Logical Operator : Logic  Operator=OR  AllPortsSameDT=off  OutDataTypeStr=boolean
  Logical Operator1 : Logic  AllPortsSameDT=off  OutDataTypeStr=boolean
  NoFail : Outport
  wires:
  FailMode/1 -> Abs/1
  Logical Operator1/1 -> NoFail/1
  Compare To Constant/1 -> Logical Operator/2
  BeforeFail/1 -> Logical Operator/1
  Abs/1 -> Compare To Constant/1
  Logical Operator/1 -> Logical Operator1/1
  FuelRemaining/1 -> Logical Operator1/2

== system Bossi_Emanuele_EE460S3D_R99/S3D_Plant/ThrusterValues/FailModes/Ufail8/MAX ==
  Action Port : ActionPort  ActionPortLabel=elseif(u1 > 0.5 & u1 < 1.5)
  Constant : Constant  Value=ULIM(Udx,2)  SampleTime=dt0
  Out1 : Outport
  wires:
  Constant/1 -> Out1/1

== system Bossi_Emanuele_EE460S3D_R99/S3D_Plant/ThrusterValues/FailModes/Ufail8/MIN ==
  Action Port : ActionPort  ActionPortLabel=if(u1 < -0.5)
  Constant : Constant  Value=ULIM(Udx,1)  SampleTime=dt0
  Out1 : Outport
  wires:
  Constant/1 -> Out1/1

== system Bossi_Emanuele_EE460S3D_R99/S3D_Plant/ThrusterValues/FailModes/Ufail9/CURRENT ==
  In1 : Inport
  Action Port : ActionPort  ActionPortLabel=else
  Out1 : Outport
  wires:
  In1/1 -> Out1/1

== system Bossi_Emanuele_EE460S3D_R99/S3D_Plant/ThrusterValues/FailModes/Ufail9/FailLogic ==
  BeforeFail : Inport
  FuelRemaining : Inport  Port=2
  FailMode : Inport  Port=3
  Abs : Abs  SaturateOnIntegerOverflow=off
  Compare To Constant : simulink/Logic and Bit Operations/Compare To Constant  relop=<=  const=0.5  OutDataTypeStr=boolean
  Logical Operator : Logic  Operator=OR  AllPortsSameDT=off  OutDataTypeStr=boolean
  Logical Operator1 : Logic  AllPortsSameDT=off  OutDataTypeStr=boolean
  NoFail : Outport
  wires:
  FailMode/1 -> Abs/1
  Logical Operator1/1 -> NoFail/1
  Compare To Constant/1 -> Logical Operator/2
  BeforeFail/1 -> Logical Operator/1
  Abs/1 -> Compare To Constant/1
  Logical Operator/1 -> Logical Operator1/1
  FuelRemaining/1 -> Logical Operator1/2

== system Bossi_Emanuele_EE460S3D_R99/S3D_Plant/ThrusterValues/FailModes/Ufail9/MAX ==
  Action Port : ActionPort  ActionPortLabel=elseif(u1 > 0.5 & u1 < 1.5)
  Constant : Constant  Value=ULIM(Udx,2)  SampleTime=dt0
  Out1 : Outport
  wires:
  Constant/1 -> Out1/1

== system Bossi_Emanuele_EE460S3D_R99/S3D_Plant/ThrusterValues/FailModes/Ufail9/MIN ==
  Action Port : ActionPort  ActionPortLabel=if(u1 < -0.5)
  Constant : Constant  Value=ULIM(Udx,1)  SampleTime=dt0
  Out1 : Outport
  wires:
  Constant/1 -> Out1/1

== system Bossi_Emanuele_EE460S3D_R99/S3D_Plant/ThrusterValues/HealthMonitoring/DetectFailures/Subsystem ==
  UCMD : Inport
  U : Inport  Port=2
  Abs : Abs  SaturateOnIntegerOverflow=off
  Compare To Constant : simulink/Logic and Bit Operations/Compare To Constant  relop=>=  const=HM_U  OutDataTypeStr=boolean
  Constant : Constant  Value=0
  Constant1 : Constant
  Logical Operator : Logic  Operator=OR  AllPortsSameDT=off  OutDataTypeStr=boolean
  Signal Specification : SignalSpecification  Dimensions=[1]
  Signal Specification1 : SignalSpecification  Dimensions=[1]
  Sum : Sum  Inputs=|+-
  Sum1 : Sum  Inputs=++|
  Switch : Switch  Criteria=u2 > Threshold  Threshold=.4  SaturateOnIntegerOverflow=off  InputSameDT=off
  Unit Delay1 : UnitDelay  SampleTime=dt0  HasFrameUpgradeWarning=on
  Unit Delay2 : UnitDelay  SampleTime=dt0  HasFrameUpgradeWarning=on
  Out1 : Outport
  wires:
  Abs/1 -> Switch/2
  Signal Specification1/1 -> Sum/2
  Signal Specification/1 -> Sum/1
  Constant/1 -> Switch/3
  Sum1/1 -> Switch/1
  Unit Delay1/1 -> Sum1/1
  Constant1/1 -> Sum1/2
  U/1 -> Signal Specification1/1
  Logical Operator/1 -> Unit Delay2/1, Out1/1
  Compare To Constant/1 -> Logical Operator/1
  Switch/1 -> Unit Delay1/1, Compare To Constant/1
  UCMD/1 -> Signal Specification/1
  Unit Delay2/1 -> Logical Operator/2
  Sum/1 -> Abs/1

== system Bossi_Emanuele_EE460S3D_R99/S3D_Plant/ThrusterValues/HealthMonitoring/DetectFailures/Subsystem1 ==
  UCMD : Inport
  U : Inport  Port=2
  Abs : Abs  SaturateOnIntegerOverflow=off
  Compare To Constant : simulink/Logic and Bit Operations/Compare To Constant  relop=>=  const=HM_U  OutDataTypeStr=boolean
  Constant : Constant  Value=0
  Constant1 : Constant
  Logical Operator : Logic  Operator=OR  AllPortsSameDT=off  OutDataTypeStr=boolean
  Signal Specification : SignalSpecification  Dimensions=[1]
  Signal Specification1 : SignalSpecification  Dimensions=[1]
  Sum : Sum  Inputs=|+-
  Sum1 : Sum  Inputs=++|
  Switch : Switch  Criteria=u2 > Threshold  Threshold=.4  SaturateOnIntegerOverflow=off  InputSameDT=off
  Unit Delay1 : UnitDelay  SampleTime=dt0  HasFrameUpgradeWarning=on
  Unit Delay2 : UnitDelay  SampleTime=dt0  HasFrameUpgradeWarning=on
  Out1 : Outport
  wires:
  Abs/1 -> Switch/2
  Signal Specification1/1 -> Sum/2
  Signal Specification/1 -> Sum/1
  Constant/1 -> Switch/3
  Sum1/1 -> Switch/1
  Unit Delay1/1 -> Sum1/1
  Constant1/1 -> Sum1/2
  U/1 -> Signal Specification1/1
  Logical Operator/1 -> Unit Delay2/1, Out1/1
  Compare To Constant/1 -> Logical Operator/1
  Switch/1 -> Unit Delay1/1, Compare To Constant/1
  UCMD/1 -> Signal Specification/1
  Unit Delay2/1 -> Logical Operator/2
  Sum/1 -> Abs/1

== system Bossi_Emanuele_EE460S3D_R99/S3D_Plant/ThrusterValues/HealthMonitoring/DetectFailures/Subsystem2 ==
  UCMD : Inport
  U : Inport  Port=2
  Abs : Abs  SaturateOnIntegerOverflow=off
  Compare To Constant : simulink/Logic and Bit Operations/Compare To Constant  relop=>=  const=HM_U  OutDataTypeStr=boolean
  Constant : Constant  Value=0
  Constant1 : Constant
  Logical Operator : Logic  Operator=OR  AllPortsSameDT=off  OutDataTypeStr=boolean
  Signal Specification : SignalSpecification  Dimensions=[1]
  Signal Specification1 : SignalSpecification  Dimensions=[1]
  Sum : Sum  Inputs=|+-
  Sum1 : Sum  Inputs=++|
  Switch : Switch  Criteria=u2 > Threshold  Threshold=.4  SaturateOnIntegerOverflow=off  InputSameDT=off
  Unit Delay1 : UnitDelay  SampleTime=dt0  HasFrameUpgradeWarning=on
  Unit Delay2 : UnitDelay  SampleTime=dt0  HasFrameUpgradeWarning=on
  Out1 : Outport
  wires:
  Abs/1 -> Switch/2
  Signal Specification1/1 -> Sum/2
  Signal Specification/1 -> Sum/1
  Constant/1 -> Switch/3
  Sum1/1 -> Switch/1
  Unit Delay1/1 -> Sum1/1
  Constant1/1 -> Sum1/2
  U/1 -> Signal Specification1/1
  Logical Operator/1 -> Unit Delay2/1, Out1/1
  Compare To Constant/1 -> Logical Operator/1
  Switch/1 -> Unit Delay1/1, Compare To Constant/1
  UCMD/1 -> Signal Specification/1
  Unit Delay2/1 -> Logical Operator/2
  Sum/1 -> Abs/1

== system Bossi_Emanuele_EE460S3D_R99/S3D_Plant/ThrusterValues/HealthMonitoring/DetectFailures/Subsystem3 ==
  UCMD : Inport
  U : Inport  Port=2
  Abs : Abs  SaturateOnIntegerOverflow=off
  Compare To Constant : simulink/Logic and Bit Operations/Compare To Constant  relop=>=  const=HM_U  OutDataTypeStr=boolean
  Constant : Constant  Value=0
  Constant1 : Constant
  Logical Operator : Logic  Operator=OR  AllPortsSameDT=off  OutDataTypeStr=boolean
  Signal Specification : SignalSpecification  Dimensions=[1]
  Signal Specification1 : SignalSpecification  Dimensions=[1]
  Sum : Sum  Inputs=|+-
  Sum1 : Sum  Inputs=++|
  Switch : Switch  Criteria=u2 > Threshold  Threshold=.4  SaturateOnIntegerOverflow=off  InputSameDT=off
  Unit Delay1 : UnitDelay  SampleTime=dt0  HasFrameUpgradeWarning=on
  Unit Delay2 : UnitDelay  SampleTime=dt0  HasFrameUpgradeWarning=on
  Out1 : Outport
  wires:
  Abs/1 -> Switch/2
  Signal Specification1/1 -> Sum/2
  Signal Specification/1 -> Sum/1
  Constant/1 -> Switch/3
  Sum1/1 -> Switch/1
  Unit Delay1/1 -> Sum1/1
  Constant1/1 -> Sum1/2
  U/1 -> Signal Specification1/1
  Logical Operator/1 -> Unit Delay2/1, Out1/1
  Compare To Constant/1 -> Logical Operator/1
  Switch/1 -> Unit Delay1/1, Compare To Constant/1
  UCMD/1 -> Signal Specification/1
  Unit Delay2/1 -> Logical Operator/2
  Sum/1 -> Abs/1

== system Bossi_Emanuele_EE460S3D_R99/S3D_Plant/ThrusterValues/HealthMonitoring/DetectFailures/Subsystem4 ==
  UCMD : Inport
  U : Inport  Port=2
  Abs : Abs  SaturateOnIntegerOverflow=off
  Compare To Constant : simulink/Logic and Bit Operations/Compare To Constant  relop=>=  const=HM_U  OutDataTypeStr=boolean
  Constant : Constant  Value=0
  Constant1 : Constant
  Logical Operator : Logic  Operator=OR  AllPortsSameDT=off  OutDataTypeStr=boolean
  Signal Specification : SignalSpecification  Dimensions=[1]
  Signal Specification1 : SignalSpecification  Dimensions=[1]
  Sum : Sum  Inputs=|+-
  Sum1 : Sum  Inputs=++|
  Switch : Switch  Criteria=u2 > Threshold  Threshold=.4  SaturateOnIntegerOverflow=off  InputSameDT=off
  Unit Delay1 : UnitDelay  SampleTime=dt0  HasFrameUpgradeWarning=on
  Unit Delay2 : UnitDelay  SampleTime=dt0  HasFrameUpgradeWarning=on
  Out1 : Outport
  wires:
  Abs/1 -> Switch/2
  Signal Specification1/1 -> Sum/2
  Signal Specification/1 -> Sum/1
  Constant/1 -> Switch/3
  Sum1/1 -> Switch/1
  Unit Delay1/1 -> Sum1/1
  Constant1/1 -> Sum1/2
  U/1 -> Signal Specification1/1
  Logical Operator/1 -> Unit Delay2/1, Out1/1
  Compare To Constant/1 -> Logical Operator/1
  Switch/1 -> Unit Delay1/1, Compare To Constant/1
  UCMD/1 -> Signal Specification/1
  Unit Delay2/1 -> Logical Operator/2
  Sum/1 -> Abs/1

== system Bossi_Emanuele_EE460S3D_R99/S3D_Plant/ThrusterValues/HealthMonitoring/DetectFailures/Subsystem5 ==
  UCMD : Inport
  U : Inport  Port=2
  Abs : Abs  SaturateOnIntegerOverflow=off
  Compare To Constant : simulink/Logic and Bit Operations/Compare To Constant  relop=>=  const=HM_U  OutDataTypeStr=boolean
  Constant : Constant  Value=0
  Constant1 : Constant
  Logical Operator : Logic  Operator=OR  AllPortsSameDT=off  OutDataTypeStr=boolean
  Signal Specification : SignalSpecification  Dimensions=[1]
  Signal Specification1 : SignalSpecification  Dimensions=[1]
  Sum : Sum  Inputs=|+-
  Sum1 : Sum  Inputs=++|
  Switch : Switch  Criteria=u2 > Threshold  Threshold=.4  SaturateOnIntegerOverflow=off  InputSameDT=off
  Unit Delay1 : UnitDelay  SampleTime=dt0  HasFrameUpgradeWarning=on
  Unit Delay2 : UnitDelay  SampleTime=dt0  HasFrameUpgradeWarning=on
  Out1 : Outport
  wires:
  Abs/1 -> Switch/2
  Signal Specification1/1 -> Sum/2
  Signal Specification/1 -> Sum/1
  Constant/1 -> Switch/3
  Sum1/1 -> Switch/1
  Unit Delay1/1 -> Sum1/1
  Constant1/1 -> Sum1/2
  U/1 -> Signal Specification1/1
  Logical Operator/1 -> Unit Delay2/1, Out1/1
  Compare To Constant/1 -> Logical Operator/1
  Switch/1 -> Unit Delay1/1, Compare To Constant/1
  UCMD/1 -> Signal Specification/1
  Unit Delay2/1 -> Logical Operator/2
  Sum/1 -> Abs/1

== system Bossi_Emanuele_EE460S3D_R99/S3D_Plant/ThrusterValues/HealthMonitoring/DetectFailures/Subsystem6 ==
  UCMD : Inport
  U : Inport  Port=2
  Abs : Abs  SaturateOnIntegerOverflow=off
  Compare To Constant : simulink/Logic and Bit Operations/Compare To Constant  relop=>=  const=HM_U  OutDataTypeStr=boolean
  Constant : Constant  Value=0
  Constant1 : Constant
  Logical Operator : Logic  Operator=OR  AllPortsSameDT=off  OutDataTypeStr=boolean
  Signal Specification : SignalSpecification  Dimensions=[1]
  Signal Specification1 : SignalSpecification  Dimensions=[1]
  Sum : Sum  Inputs=|+-
  Sum1 : Sum  Inputs=++|
  Switch : Switch  Criteria=u2 > Threshold  Threshold=.4  SaturateOnIntegerOverflow=off  InputSameDT=off
  Unit Delay1 : UnitDelay  SampleTime=dt0  HasFrameUpgradeWarning=on
  Unit Delay2 : UnitDelay  SampleTime=dt0  HasFrameUpgradeWarning=on
  Out1 : Outport
  wires:
  Abs/1 -> Switch/2
  Signal Specification1/1 -> Sum/2
  Signal Specification/1 -> Sum/1
  Constant/1 -> Switch/3
  Sum1/1 -> Switch/1
  Unit Delay1/1 -> Sum1/1
  Constant1/1 -> Sum1/2
  U/1 -> Signal Specification1/1
  Logical Operator/1 -> Unit Delay2/1, Out1/1
  Compare To Constant/1 -> Logical Operator/1
  Switch/1 -> Unit Delay1/1, Compare To Constant/1
  UCMD/1 -> Signal Specification/1
  Unit Delay2/1 -> Logical Operator/2
  Sum/1 -> Abs/1

== system Bossi_Emanuele_EE460S3D_R99/S3D_Plant/ThrusterValues/HealthMonitoring/DetectFailures/Subsystem7 ==
  UCMD : Inport
  U : Inport  Port=2
  Abs : Abs  SaturateOnIntegerOverflow=off
  Compare To Constant : simulink/Logic and Bit Operations/Compare To Constant  relop=>=  const=HM_U  OutDataTypeStr=boolean
  Constant : Constant  Value=0
  Constant1 : Constant
  Logical Operator : Logic  Operator=OR  AllPortsSameDT=off  OutDataTypeStr=boolean
  Signal Specification : SignalSpecification  Dimensions=[1]
  Signal Specification1 : SignalSpecification  Dimensions=[1]
  Sum : Sum  Inputs=|+-
  Sum1 : Sum  Inputs=++|
  Switch : Switch  Criteria=u2 > Threshold  Threshold=.4  SaturateOnIntegerOverflow=off  InputSameDT=off
  Unit Delay1 : UnitDelay  SampleTime=dt0  HasFrameUpgradeWarning=on
  Unit Delay2 : UnitDelay  SampleTime=dt0  HasFrameUpgradeWarning=on
  Out1 : Outport
  wires:
  Abs/1 -> Switch/2
  Signal Specification1/1 -> Sum/2
  Signal Specification/1 -> Sum/1
  Constant/1 -> Switch/3
  Sum1/1 -> Switch/1
  Unit Delay1/1 -> Sum1/1
  Constant1/1 -> Sum1/2
  U/1 -> Signal Specification1/1
  Logical Operator/1 -> Unit Delay2/1, Out1/1
  Compare To Constant/1 -> Logical Operator/1
  Switch/1 -> Unit Delay1/1, Compare To Constant/1
  UCMD/1 -> Signal Specification/1
  Unit Delay2/1 -> Logical Operator/2
  Sum/1 -> Abs/1

== system Bossi_Emanuele_EE460S3D_R99/S3D_Plant/ThrusterValues/HealthMonitoring/DetectFailures/Subsystem8 ==
  UCMD : Inport
  U : Inport  Port=2
  Abs : Abs  SaturateOnIntegerOverflow=off
  Compare To Constant : simulink/Logic and Bit Operations/Compare To Constant  relop=>=  const=HM_U  OutDataTypeStr=boolean
  Constant : Constant  Value=0
  Constant1 : Constant
  Logical Operator : Logic  Operator=OR  AllPortsSameDT=off  OutDataTypeStr=boolean
  Signal Specification : SignalSpecification  Dimensions=[1]
  Signal Specification1 : SignalSpecification  Dimensions=[1]
  Sum : Sum  Inputs=|+-
  Sum1 : Sum  Inputs=++|
  Switch : Switch  Criteria=u2 > Threshold  Threshold=.4  SaturateOnIntegerOverflow=off  InputSameDT=off
  Unit Delay1 : UnitDelay  SampleTime=dt0  HasFrameUpgradeWarning=on
  Unit Delay2 : UnitDelay  SampleTime=dt0  HasFrameUpgradeWarning=on
  Out1 : Outport
  wires:
  Abs/1 -> Switch/2
  Signal Specification1/1 -> Sum/2
  Signal Specification/1 -> Sum/1
  Constant/1 -> Switch/3
  Sum1/1 -> Switch/1
  Unit Delay1/1 -> Sum1/1
  Constant1/1 -> Sum1/2
  U/1 -> Signal Specification1/1
  Logical Operator/1 -> Unit Delay2/1, Out1/1
  Compare To Constant/1 -> Logical Operator/1
  Switch/1 -> Unit Delay1/1, Compare To Constant/1
  UCMD/1 -> Signal Specification/1
  Unit Delay2/1 -> Logical Operator/2
  Sum/1 -> Abs/1
